simulink model "DualBuckPPS_PI"  (R2024b)
settings: Solver=ode45  StartTime=0.0  StopTime=0.8  RelTol=1e-3
model workspace (MAT data in the model file):
  D = 50
  T = 0.033
  T_pulse = 0.02
undefined symbols (not defined in the file): I_I, I_V, P, P_I, P_V, TP
libraries: spsOnDelayLib x13, spsCurrentMeasurementLib x11, spsSeriesRLCBranchLib x7, dspfdesign x6, spsMosfetLib x4, slpidlib x4, spsVoltageMeasurementLib x4, simulink x3, spsControlledCurrentSourceLib x1, spsDCVoltageSourceLib x1, spspowerguiLib x1
settings Model: SimulationMode=accelerator  Creator=10474  LastModifiedBy=admin
settings SolverCC: AlgebraicLoopSolver=TrustRegion
settings OptimizationCC: ReuseModelBlockBuffer=off
settings DebuggingCC: UnconnectedInputMsg=warning  UnconnectedOutputMsg=warning  UnconnectedLineMsg=warning  ArithmeticOperatorsInVariantConditions=warning
settings ModelReferenceCC: EnableRefExpFcnMdlSchedulingChecks=on
settings SFSimCC: CustomCodeUndefinedFunction=UseInterfaceOnly
settings RTWCC: GPUComputeCapability=3.5
settings CodeAppCC: StateflowObjectComments=on

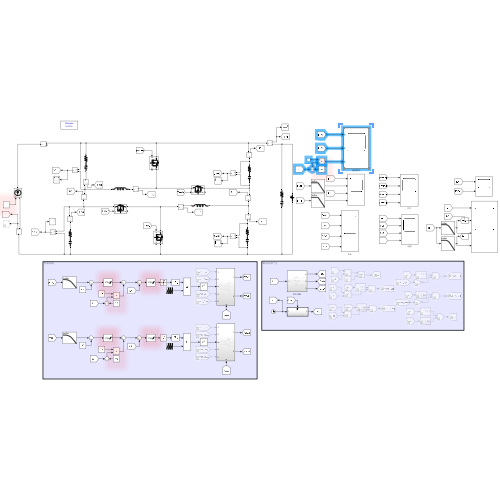
[thumbnail: Simulink's stored preview of the top-level diagram]
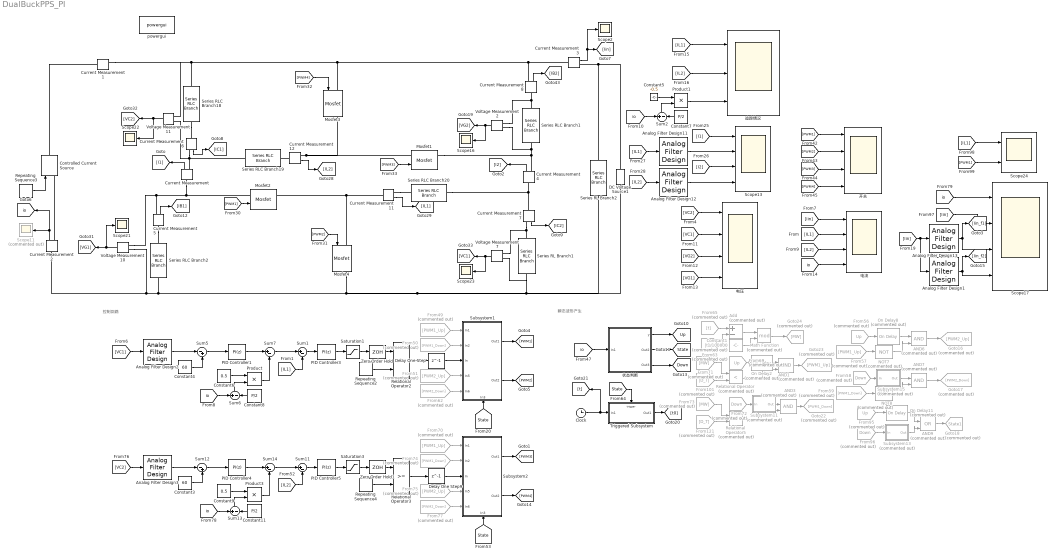
== system DualBuckPPS_PI ==
  note: 控制回路
  note: 瞬态波形产生
  AND{1,3,6..7} (4 alike) : Logic  Commented=on  IconShape=distinctive  AllPortsSameDT=off  OutDataTypeStr=boolean
  AND9 : Logic  Commented=on  Operator=OR  IconShape=distinctive  AllPortsSameDT=off  OutDataTypeStr=boolean
  Add : Sum  Commented=on  Inputs=+-
  Analog Filter Design1 : dspfdesign/Analog Filter Design  method=Butterworth  filttype=Lowpass  N=2  Wlo=2*pi*2500  Whi=80  Rp=2  Rs=40
  Analog Filter Design11 : dspfdesign/Analog Filter Design  method=Butterworth  filttype=Lowpass  N=8  Wlo=2*pi*5000  Whi=80  Rp=2  Rs=40
  Analog Filter Design12 : dspfdesign/Analog Filter Design  method=Butterworth  filttype=Lowpass  N=8  Wlo=2*pi*5000  Whi=80  Rp=2  Rs=40
  Analog Filter Design13 : dspfdesign/Analog Filter Design  method=Butterworth  filttype=Lowpass  N=2  Wlo=2*pi*10000  Whi=80  Rp=2  Rs=40
  Analog Filter Design2 : dspfdesign/Analog Filter Design  method=Butterworth  filttype=Lowpass  N=1  Wlo=10  Whi=80  Rp=2  Rs=40
  Analog Filter Design3 : dspfdesign/Analog Filter Design  method=Butterworth  filttype=Lowpass  N=1  Wlo=10  Whi=80  Rp=2  Rs=40
  Clock : Clock
  Constant1 : Constant  Commented=on  Value=1/100000
  Constant11 : Constant  Value=P/2
  Constant3 : Constant  Value=60
  Constant4 : Constant  Value=60
  Constant5 : Constant  Value=-0.5
  Constant6 : Constant  Value=0.5
  Constant7 : Constant  Value=P/2
  Constant8 : Constant  Value=P/2
  Constant9 : Constant  Value=0.5
  Controlled Current Source : spsControlledCurrentSourceLib/Controlled Current Source  Initialize=on  Source_Type=DC  Amplitude=0  Phase=0  Frequency=0  Measurements=None
  Current Measurement{,1..8,11..12} (11 alike) : spsCurrentMeasurementLib/Current Measurement  PhasorSimulation=off  OutputType=Complex  PSBequivalent=0
  DC Voltage Source1 : spsDCVoltageSourceLib/DC Voltage Source  Amplitude=270  Measurements=None
  Delay One Step : Delay  DelayLength=1
  Delay One Step9 : Delay  DelayLength=1
  From101 : From  Commented=on  GotoTag=D_T
  From121 : From  Commented=on  GotoTag=D_T
  From49 : From  Commented=on  GotoTag=PWM1_Up
  From50 : From  Commented=on  GotoTag=PWM1_Down
  From51 : From  Commented=on  GotoTag=PWM2_Up
  From56 : From  Commented=on  GotoTag=Up  TagVisibility=global
  From57 : From  Commented=on  GotoTag=PWM1_Up
  From58 : From  Commented=on  GotoTag=Down  TagVisibility=global
  From59 : From  Commented=on  GotoTag=PWM1_Down
  From62 : From  Commented=on  GotoTag=PWM2_Down
  From63 : From  Commented=on  GotoTag=t0
  From65 : From  Commented=on  GotoTag=t
  From69 : From  Commented=on  GotoTag=Up  TagVisibility=global
  From70 : From  Commented=on  GotoTag=PWM1_Up
  From71 : From  Commented=on  GotoTag=MW
  From72 : From  Commented=on  GotoTag=Down  TagVisibility=global
  From73 : From  Commented=on  GotoTag=MW
  From74 : From  Commented=on  GotoTag=PWM1_Down
  From75 : From  Commented=on  GotoTag=PWM2_Up
  From77 : From  Commented=on  GotoTag=PWM2_Down
  From95 : From  Commented=on  GotoTag=Up  TagVisibility=global
  From96 : From  Commented=on  GotoTag=Down  TagVisibility=global
  Goto16 : Goto  Commented=on  GotoTag=PWM2_Up
  Goto17 : Goto  Commented=on  GotoTag=PWM2_Down
  Goto18 : Goto  Commented=on  GotoTag=State1  TagVisibility=global
  Goto22 : Goto  Commented=on  GotoTag=PWM1_Down
  Goto23 : Goto  Commented=on  GotoTag=PWM1_Up
  Goto24 : Goto  Commented=on  GotoTag=MW
  Math Function : Math  Commented=on  Operator=mod
  Mosfet{1..4} (4 alike) : spsMosfetLib/Mosfet  Ron=53e-3  Lon=0  Rd=0.001  Vfd=2  IC=0  Rs=1e5  Cs=inf  Measurements=on
  NOT7 : Logic  Commented=on  Operator=NOT  IconShape=distinctive  AllPortsSameDT=off  OutDataTypeStr=boolean
  NOT8 : Logic  Commented=on  Operator=NOT  IconShape=distinctive  AllPortsSameDT=off  OutDataTypeStr=boolean
  On Delay11 : spsOnDelayLib/On Delay  Commented=on  DelayType=Off delay  delay=ceil(TP*1e5)*1e-5-TP  ic=0  Ts=0
  On Delay2 : spsOnDelayLib/On Delay  Commented=on  DelayType=Off delay  delay=ceil(TP*1e5)*1e-5-TP  ic=0  Ts=0
  On Delay8 : spsOnDelayLib/On Delay  Commented=on  DelayType=Off delay  delay=ceil(TP*1e5)*1e-5-TP  ic=0  Ts=0
  PID Controller1 : slpidlib/PID Controller  Controller=PI  Form=Parallel  TimeDomain=Discrete-time  UseExternalTs=off  SampleTime=-1  IntegratorMethod=Forward Euler  FilterMethod=Forward Euler  ControllerParametersSource=internal  P=P_V  I=I_V  UseKiTs=off  D=0  UseExternalDerivativeSource=off  N=100  UseFilter=on  TunerSelectOption=Transfer Function Based (PID Tuner App)  InitialConditionSource=internal  InitialConditionForIntegrator=0  InitialConditionForFilter=0  DifferentiatorICPrevScaledInput=0  ExternalReset=none  TrackingMode=off  Kt=1  LimitOutput=on  SatLimitsSource=internal  UpperSaturationLimit=10  LowerSaturationLimit=-10  LinearizeAsGain=on  AntiWindupMode=none  Kb=1  LimitIntegrator=off  UpperIntegratorSaturationLimit=inf  LowerIntegratorSaturationLimit=-inf  POutMin=[]  POutMax=[]  IOutMin=[]  IOutMax=[]  DOutMin=[]  DOutMax=[]  NOutMin=[]  NOutMax=[]  SumOutMin=[]  SumOutMax=[]  SaturationOutMin=[]  SaturationOutMax=[]  PParamMin=[]  PParamMax=[]  IParamMin=[]  IParamMax=[]  DParamMin=[]  DParamMax=[]  NParamMin=[]  NParamMax=[]  KbParamMin=[]  KbParamMax=[]  KtParamMin=[]  KtParamMax=[]  KbOutMin=[]  KbOutMax=[]  KtOutMin=[]  KtOutMax=[]  IntegratorOutMin=[]  IntegratorOutMax=[]  FilterOutMin=[]  FilterOutMax=[]  SumI1OutMin=[]  SumI1OutMax=[]  SumI2OutMin=[]  SumI2OutMax=[]  SumI3OutMin=[]  SumI3OutMax=[]  SumI4OutMin=[]  SumI4OutMax=[]  SumDOutMin=[]  SumDOutMax=[]  DifferentiatorOutMin=[]  DifferentiatorOutMax=[]  FilterDiffOutCoefMin=[]  FilterDiffOutCoefMax=[]  ReciprocalOutMin=[]  ReciprocalOutMax=[]  SumDenOutMin=[]  SumDenOutMax=[]  SumNumOutMin=[]  SumNumOutMax=[]  DivideOutMin=[]  DivideOutMax=[]  UdiffTsProdOutMin=[]  UdiffTsProdOutMax=[]  NTsProdOutMin=[]  NTsProdOutMax=[]  UintegralTsProdOutMin=[]  UintegralTsProdOutMax=[]  UngainTsProdOutMin=[]  UngainTsProdOutMax=[]  ClampingZeroOutDataTypeStr=Inherit: Inherit via back propagation  ClampingZeroOutMin=[]  ClampingZeroOutMax=[]  FilterDenConstantOutDataTypeStr=Inherit: Inherit via back propagation  FilterDenConstantOutMin=[]  FilterDenConstantOutMax=[]  PCopyOutDataTypeStr=Inherit: Inherit via back propagation  PCopyOutMin=[]  PCopyOutMax=[]  NCopyOutDataTypeStr=Inherit: Inherit via back propagation  NCopyOutMin=[]  NCopyOutMax=[]  IntegratorContinuousStateAttributes=''  IntegratorStateMustResolveToSignalObject=off  IntegratorRTWStateStorageClass=Auto  FilterContinuousStateAttributes=''  FilterStateMustResolveToSignalObject=off  FilterRTWStateStorageClass=Auto  ParallelPVariant=InternalParameters  IdealPVariant=Disabled  IVariant=InternalParameters  DVariant=Disabled  IntegratorVariant=Discrete  SatVariant=Enabled  AWVariant=Passthrough  PCopyVariant=Disabled  TRVariant=Disabled  FdbkBlocksVariant=Forward  IdealPFdbkVariant=Disabled  SatFdbkVariant=Disabled  DerivativeFilterVariant=Disabled  NVariant=Disabled  NCopyVariant=Disabled_SignalSpec  FilterICVariant=Disabled  IntegratorICVariant=InternalICs  ExternalResetVariant=Disabled  TRSumVariant=Passthrough  SumFdbkVariant=Disabled  SumVariant=Sum_PI  TsampFilterVariant=InternalTs  TsampNgainVariant=Passthrough  TsampIntegralVariant=Disabled_SignalSpec  ExternalSaturationOutDataTypeStr=Inherit: Same as second input  DerivativeSourceVariant=Disabled  PreIntVariant=InternalPreInt
  PID Controller3 : slpidlib/PID Controller  Controller=PI  Form=Parallel  TimeDomain=Discrete-time  UseExternalTs=off  SampleTime=-1  IntegratorMethod=Forward Euler  FilterMethod=Forward Euler  ControllerParametersSource=internal  P=P_I  I=I_I  UseKiTs=off  D=0  UseExternalDerivativeSource=off  N=100  UseFilter=on  TunerSelectOption=Transfer Function Based (PID Tuner App)  InitialConditionSource=internal  InitialConditionForIntegrator=0  InitialConditionForFilter=0  DifferentiatorICPrevScaledInput=0  ExternalReset=none  TrackingMode=off  Kt=1  LimitOutput=on  SatLimitsSource=internal  UpperSaturationLimit=0.98  LowerSaturationLimit=0  LinearizeAsGain=on  AntiWindupMode=none  Kb=1  LimitIntegrator=off  UpperIntegratorSaturationLimit=inf  LowerIntegratorSaturationLimit=-inf  POutMin=[]  POutMax=[]  IOutMin=[]  IOutMax=[]  DOutMin=[]  DOutMax=[]  NOutMin=[]  NOutMax=[]  SumOutMin=[]  SumOutMax=[]  SaturationOutMin=[]  SaturationOutMax=[]  PParamMin=[]  PParamMax=[]  IParamMin=[]  IParamMax=[]  DParamMin=[]  DParamMax=[]  NParamMin=[]  NParamMax=[]  KbParamMin=[]  KbParamMax=[]  KtParamMin=[]  KtParamMax=[]  KbOutMin=[]  KbOutMax=[]  KtOutMin=[]  KtOutMax=[]  IntegratorOutMin=[]  IntegratorOutMax=[]  FilterOutMin=[]  FilterOutMax=[]  SumI1OutMin=[]  SumI1OutMax=[]  SumI2OutMin=[]  SumI2OutMax=[]  SumI3OutMin=[]  SumI3OutMax=[]  SumI4OutMin=[]  SumI4OutMax=[]  SumDOutMin=[]  SumDOutMax=[]  DifferentiatorOutMin=[]  DifferentiatorOutMax=[]  FilterDiffOutCoefMin=[]  FilterDiffOutCoefMax=[]  ReciprocalOutMin=[]  ReciprocalOutMax=[]  SumDenOutMin=[]  SumDenOutMax=[]  SumNumOutMin=[]  SumNumOutMax=[]  DivideOutMin=[]  DivideOutMax=[]  UdiffTsProdOutMin=[]  UdiffTsProdOutMax=[]  NTsProdOutMin=[]  NTsProdOutMax=[]  UintegralTsProdOutMin=[]  UintegralTsProdOutMax=[]  UngainTsProdOutMin=[]  UngainTsProdOutMax=[]  ClampingZeroOutDataTypeStr=Inherit: Inherit via back propagation  ClampingZeroOutMin=[]  ClampingZeroOutMax=[]  FilterDenConstantOutDataTypeStr=Inherit: Inherit via back propagation  FilterDenConstantOutMin=[]  FilterDenConstantOutMax=[]  PCopyOutDataTypeStr=Inherit: Inherit via back propagation  PCopyOutMin=[]  PCopyOutMax=[]  NCopyOutDataTypeStr=Inherit: Inherit via back propagation  NCopyOutMin=[]  NCopyOutMax=[]  IntegratorContinuousStateAttributes=''  IntegratorStateMustResolveToSignalObject=off  IntegratorRTWStateStorageClass=Auto  FilterContinuousStateAttributes=''  FilterStateMustResolveToSignalObject=off  FilterRTWStateStorageClass=Auto  ParallelPVariant=InternalParameters  IdealPVariant=Disabled  IVariant=InternalParameters  DVariant=Disabled  IntegratorVariant=Discrete  SatVariant=Enabled  AWVariant=Passthrough  PCopyVariant=Disabled  TRVariant=Disabled  FdbkBlocksVariant=Forward  IdealPFdbkVariant=Disabled  SatFdbkVariant=Disabled  DerivativeFilterVariant=Disabled  NVariant=Disabled  NCopyVariant=Disabled_SignalSpec  FilterICVariant=Disabled  IntegratorICVariant=InternalICs  ExternalResetVariant=Disabled  TRSumVariant=Passthrough  SumFdbkVariant=Disabled  SumVariant=Sum_PI  TsampFilterVariant=InternalTs  TsampNgainVariant=Passthrough  TsampIntegralVariant=Disabled_SignalSpec  ExternalSaturationOutDataTypeStr=Inherit: Same as second input  DerivativeSourceVariant=Disabled  PreIntVariant=InternalPreInt
  PID Controller4 : slpidlib/PID Controller  Controller=PI  Form=Parallel  TimeDomain=Discrete-time  UseExternalTs=off  SampleTime=-1  IntegratorMethod=Forward Euler  FilterMethod=Forward Euler  ControllerParametersSource=internal  P=P_V  I=I_V  UseKiTs=off  D=0  UseExternalDerivativeSource=off  N=100  UseFilter=on  TunerSelectOption=Transfer Function Based (PID Tuner App)  InitialConditionSource=internal  InitialConditionForIntegrator=0  InitialConditionForFilter=0  DifferentiatorICPrevScaledInput=0  ExternalReset=none  TrackingMode=off  Kt=1  LimitOutput=on  SatLimitsSource=internal  UpperSaturationLimit=10  LowerSaturationLimit=-10  LinearizeAsGain=on  AntiWindupMode=none  Kb=1  LimitIntegrator=off  UpperIntegratorSaturationLimit=inf  LowerIntegratorSaturationLimit=-inf  POutMin=[]  POutMax=[]  IOutMin=[]  IOutMax=[]  DOutMin=[]  DOutMax=[]  NOutMin=[]  NOutMax=[]  SumOutMin=[]  SumOutMax=[]  SaturationOutMin=[]  SaturationOutMax=[]  PParamMin=[]  PParamMax=[]  IParamMin=[]  IParamMax=[]  DParamMin=[]  DParamMax=[]  NParamMin=[]  NParamMax=[]  KbParamMin=[]  KbParamMax=[]  KtParamMin=[]  KtParamMax=[]  KbOutMin=[]  KbOutMax=[]  KtOutMin=[]  KtOutMax=[]  IntegratorOutMin=[]  IntegratorOutMax=[]  FilterOutMin=[]  FilterOutMax=[]  SumI1OutMin=[]  SumI1OutMax=[]  SumI2OutMin=[]  SumI2OutMax=[]  SumI3OutMin=[]  SumI3OutMax=[]  SumI4OutMin=[]  SumI4OutMax=[]  SumDOutMin=[]  SumDOutMax=[]  DifferentiatorOutMin=[]  DifferentiatorOutMax=[]  FilterDiffOutCoefMin=[]  FilterDiffOutCoefMax=[]  ReciprocalOutMin=[]  ReciprocalOutMax=[]  SumDenOutMin=[]  SumDenOutMax=[]  SumNumOutMin=[]  SumNumOutMax=[]  DivideOutMin=[]  DivideOutMax=[]  UdiffTsProdOutMin=[]  UdiffTsProdOutMax=[]  NTsProdOutMin=[]  NTsProdOutMax=[]  UintegralTsProdOutMin=[]  UintegralTsProdOutMax=[]  UngainTsProdOutMin=[]  UngainTsProdOutMax=[]  ClampingZeroOutDataTypeStr=Inherit: Inherit via back propagation  ClampingZeroOutMin=[]  ClampingZeroOutMax=[]  FilterDenConstantOutDataTypeStr=Inherit: Inherit via back propagation  FilterDenConstantOutMin=[]  FilterDenConstantOutMax=[]  PCopyOutDataTypeStr=Inherit: Inherit via back propagation  PCopyOutMin=[]  PCopyOutMax=[]  NCopyOutDataTypeStr=Inherit: Inherit via back propagation  NCopyOutMin=[]  NCopyOutMax=[]  IntegratorContinuousStateAttributes=''  IntegratorStateMustResolveToSignalObject=off  IntegratorRTWStateStorageClass=Auto  FilterContinuousStateAttributes=''  FilterStateMustResolveToSignalObject=off  FilterRTWStateStorageClass=Auto  ParallelPVariant=InternalParameters  IdealPVariant=Disabled  IVariant=InternalParameters  DVariant=Disabled  IntegratorVariant=Discrete  SatVariant=Enabled  AWVariant=Passthrough  PCopyVariant=Disabled  TRVariant=Disabled  FdbkBlocksVariant=Forward  IdealPFdbkVariant=Disabled  SatFdbkVariant=Disabled  DerivativeFilterVariant=Disabled  NVariant=Disabled  NCopyVariant=Disabled_SignalSpec  FilterICVariant=Disabled  IntegratorICVariant=InternalICs  ExternalResetVariant=Disabled  TRSumVariant=Passthrough  SumFdbkVariant=Disabled  SumVariant=Sum_PI  TsampFilterVariant=InternalTs  TsampNgainVariant=Passthrough  TsampIntegralVariant=Disabled_SignalSpec  ExternalSaturationOutDataTypeStr=Inherit: Same as second input  DerivativeSourceVariant=Disabled  PreIntVariant=InternalPreInt
  PID Controller5 : slpidlib/PID Controller  Controller=PI  Form=Parallel  TimeDomain=Discrete-time  UseExternalTs=off  SampleTime=-1  IntegratorMethod=Forward Euler  FilterMethod=Forward Euler  ControllerParametersSource=internal  P=P_I  I=I_I  UseKiTs=off  D=0  UseExternalDerivativeSource=off  N=100  UseFilter=on  TunerSelectOption=Transfer Function Based (PID Tuner App)  InitialConditionSource=internal  InitialConditionForIntegrator=0  InitialConditionForFilter=0  DifferentiatorICPrevScaledInput=0  ExternalReset=none  TrackingMode=off  Kt=1  LimitOutput=on  SatLimitsSource=internal  UpperSaturationLimit=0.98  LowerSaturationLimit=0  LinearizeAsGain=on  AntiWindupMode=none  Kb=1  LimitIntegrator=off  UpperIntegratorSaturationLimit=inf  LowerIntegratorSaturationLimit=-inf  POutMin=[]  POutMax=[]  IOutMin=[]  IOutMax=[]  DOutMin=[]  DOutMax=[]  NOutMin=[]  NOutMax=[]  SumOutMin=[]  SumOutMax=[]  SaturationOutMin=[]  SaturationOutMax=[]  PParamMin=[]  PParamMax=[]  IParamMin=[]  IParamMax=[]  DParamMin=[]  DParamMax=[]  NParamMin=[]  NParamMax=[]  KbParamMin=[]  KbParamMax=[]  KtParamMin=[]  KtParamMax=[]  KbOutMin=[]  KbOutMax=[]  KtOutMin=[]  KtOutMax=[]  IntegratorOutMin=[]  IntegratorOutMax=[]  FilterOutMin=[]  FilterOutMax=[]  SumI1OutMin=[]  SumI1OutMax=[]  SumI2OutMin=[]  SumI2OutMax=[]  SumI3OutMin=[]  SumI3OutMax=[]  SumI4OutMin=[]  SumI4OutMax=[]  SumDOutMin=[]  SumDOutMax=[]  DifferentiatorOutMin=[]  DifferentiatorOutMax=[]  FilterDiffOutCoefMin=[]  FilterDiffOutCoefMax=[]  ReciprocalOutMin=[]  ReciprocalOutMax=[]  SumDenOutMin=[]  SumDenOutMax=[]  SumNumOutMin=[]  SumNumOutMax=[]  DivideOutMin=[]  DivideOutMax=[]  UdiffTsProdOutMin=[]  UdiffTsProdOutMax=[]  NTsProdOutMin=[]  NTsProdOutMax=[]  UintegralTsProdOutMin=[]  UintegralTsProdOutMax=[]  UngainTsProdOutMin=[]  UngainTsProdOutMax=[]  ClampingZeroOutDataTypeStr=Inherit: Inherit via back propagation  ClampingZeroOutMin=[]  ClampingZeroOutMax=[]  FilterDenConstantOutDataTypeStr=Inherit: Inherit via back propagation  FilterDenConstantOutMin=[]  FilterDenConstantOutMax=[]  PCopyOutDataTypeStr=Inherit: Inherit via back propagation  PCopyOutMin=[]  PCopyOutMax=[]  NCopyOutDataTypeStr=Inherit: Inherit via back propagation  NCopyOutMin=[]  NCopyOutMax=[]  IntegratorContinuousStateAttributes=''  IntegratorStateMustResolveToSignalObject=off  IntegratorRTWStateStorageClass=Auto  FilterContinuousStateAttributes=''  FilterStateMustResolveToSignalObject=off  FilterRTWStateStorageClass=Auto  ParallelPVariant=InternalParameters  IdealPVariant=Disabled  IVariant=InternalParameters  DVariant=Disabled  IntegratorVariant=Discrete  SatVariant=Enabled  AWVariant=Passthrough  PCopyVariant=Disabled  TRVariant=Disabled  FdbkBlocksVariant=Forward  IdealPFdbkVariant=Disabled  SatFdbkVariant=Disabled  DerivativeFilterVariant=Disabled  NVariant=Disabled  NCopyVariant=Disabled_SignalSpec  FilterICVariant=Disabled  IntegratorICVariant=InternalICs  ExternalResetVariant=Disabled  TRSumVariant=Passthrough  SumFdbkVariant=Disabled  SumVariant=Sum_PI  TsampFilterVariant=InternalTs  TsampNgainVariant=Passthrough  TsampIntegralVariant=Disabled_SignalSpec  ExternalSaturationOutDataTypeStr=Inherit: Same as second input  DerivativeSourceVariant=Disabled  PreIntVariant=InternalPreInt
  Product : Product
  Product1 : Product
  Product3 : Product
  Relational Operator : RelationalOperator  Commented=on  Operator=<  OutDataTypeStr=boolean  RndMeth=Simplest  InputSameDT=off
  Relational Operator2 : RelationalOperator  OutDataTypeStr=boolean  RndMeth=Simplest  InputSameDT=off
  Relational Operator3 : RelationalOperator  OutDataTypeStr=boolean  RndMeth=Simplest  InputSameDT=off
  Relational Operator5 : RelationalOperator  Commented=on  Operator=<  OutDataTypeStr=boolean  RndMeth=Simplest  InputSameDT=off
  Repeating Sequence2 : simulink/Sources/Repeating Sequence  rep_seq_t=[0 1/100000]  rep_seq_y=[0 1]
  Repeating Sequence3 : simulink/Sources/Repeating Sequence  rep_seq_t=[0 TP T_pulse/2+TP T_pulse/2+2*TP T_pulse]  rep_seq_y=[0 P P 0 0]
  Repeating Sequence4 : simulink/Sources/Repeating Sequence  rep_seq_t=[0 1/100000]  rep_seq_y=[0 1]
  Saturation1 : Saturate  UpperLimit=0.98  LowerLimit=0
  Saturation3 : Saturate  UpperLimit=0.98  LowerLimit=0
  Scope11 : Scope  Commented=on
  Scope13 : Scope  NumInputPorts=4
  Scope{2,16,21..23} (5 alike) : Scope
  Scope17 : Scope  NumInputPorts=4
  Scope24 : Scope  NumInputPorts=2
  Series RL Branch1 : spsSeriesRLCBranchLib/Series RLC Branch  LConnTagsString=__new0  RConnTagsString=__new0  BranchType=RC  Resistance=0.001  Inductance=1e-3  SetiL0=off  InitialCurrent=0  Capacitance=1e-6  Setx0=on  InitialVoltage=12  Measurements=None
  Series RL Branch2 : spsSeriesRLCBranchLib/Series RLC Branch  LConnTagsString=__new0  RConnTagsString=__new0  BranchType=RC  Resistance=0.001  Inductance=1e-3  SetiL0=off  InitialCurrent=0  Capacitance=100e-6  Setx0=on  InitialVoltage=270  Measurements=None
  Series RLC Branch1 : spsSeriesRLCBranchLib/Series RLC Branch  LConnTagsString=__new0  RConnTagsString=__new0  BranchType=RC  Resistance=0.001  Inductance=1e-3  SetiL0=off  InitialCurrent=0  Capacitance=2.48e-3  Setx0=on  InitialVoltage=12  Measurements=None
  Series RLC Branch18 : spsSeriesRLCBranchLib/Series RLC Branch  LConnTagsString=__new0  RConnTagsString=__new0  BranchType=RC  Resistance=0.001  Inductance=1e-3  SetiL0=off  InitialCurrent=0  Capacitance=1e-6  Setx0=on  InitialVoltage=12  Measurements=None
  Series RLC Branch19 : spsSeriesRLCBranchLib/Series RLC Branch  LConnTagsString=__new0  RConnTagsString=__new0  BranchType=L  Resistance=0.01  Inductance=260e-6  SetiL0=off  InitialCurrent=15  Capacitance=1e-3  Setx0=off  InitialVoltage=0  Measurements=None
  Series RLC Branch2 : spsSeriesRLCBranchLib/Series RLC Branch  LConnTagsString=__new0  RConnTagsString=__new0  BranchType=RC  Resistance=0.2  Inductance=1e-3  SetiL0=off  InitialCurrent=0  Capacitance=2.48e-3  Setx0=on  InitialVoltage=12  Measurements=None
  Series RLC Branch20 : spsSeriesRLCBranchLib/Series RLC Branch  LConnTagsString=__new0  RConnTagsString=__new0  BranchType=L  Resistance=0.01  Inductance=260e-6  SetiL0=off  InitialCurrent=5  Capacitance=1e-3  Setx0=off  InitialVoltage=0  Measurements=None
  Subsystem1 : Subsystem
      settings: PortSchema="{\"entries\":[{\"content\":{\"sides\":[{\"content\":{\"connectorIds\":[\"In1\",\"In2\",\"In3\",\"In4\",\"In5\"]},\"type\":\"ConnectorPlacement.EquallySpacedRectSide\",\"uuid\":\"12f56cea-dd87-479d-8ac5-f677a0a856ab\"},{\"content\":{\"connectorIds\":[\"Out1\",\"Out2\"],\"side\":\"RIGHT\"},\"type\":\"ConnectorPlacement.EquallySpacedRectSide\",\"uuid\":\"93daadb0-c8ef-4d9e-87ae-a550f970c223\"},{\"content\":{\"side\":\"TOP\"},\"type\":\"ConnectorPlacement.EquallySpacedRectSide\",\"uuid\":\"18f26d28-3d48-45f0-84e1-51e7663a8b99\"},{\"content\":{\"connectorIds\":[\"In6\"],\"side\":\"BOTTOM\"},\"type\":\"ConnectorPlacement.EquallySpacedRectSide\",\"uuid\":\"53ae5f66-9a34-49e2-9ad8-502cdcf805c1\"}]},\"type\":\"ConnectorPlacement.EquallySpacedConnector\",\"uuid\":\"751889f7-46a5-4d64-ba57-d2d7ffe777e8\"}],\"packageUris\":[\"http://schema.mathworks.com/mf0/Connector/R2020b\"],\"version\":\"1.0\"}"
  Subsystem11 : Subsystem  Commented=on
  Subsystem13 : Subsystem  Commented=on
  Subsystem15 : Subsystem  Commented=on
  Subsystem2 : Subsystem
      settings: PortSchema="{\"entries\":[{\"content\":{\"sides\":[{\"content\":{\"connectorIds\":[\"In1\",\"In2\",\"In3\",\"In4\",\"In5\"]},\"type\":\"ConnectorPlacement.EquallySpacedRectSide\",\"uuid\":\"12f56cea-dd87-479d-8ac5-f677a0a856ab\"},{\"content\":{\"connectorIds\":[\"Out1\",\"Out2\"],\"side\":\"RIGHT\"},\"type\":\"ConnectorPlacement.EquallySpacedRectSide\",\"uuid\":\"93daadb0-c8ef-4d9e-87ae-a550f970c223\"},{\"content\":{\"side\":\"TOP\"},\"type\":\"ConnectorPlacement.EquallySpacedRectSide\",\"uuid\":\"18f26d28-3d48-45f0-84e1-51e7663a8b99\"},{\"content\":{\"connectorIds\":[\"In6\"],\"side\":\"BOTTOM\"},\"type\":\"ConnectorPlacement.EquallySpacedRectSide\",\"uuid\":\"53ae5f66-9a34-49e2-9ad8-502cdcf805c1\"}]},\"type\":\"ConnectorPlacement.EquallySpacedConnector\",\"uuid\":\"751889f7-46a5-4d64-ba57-d2d7ffe777e8\"}],\"packageUris\":[\"http://schema.mathworks.com/mf0/Connector/R2020b\"],\"version\":\"1.0\"}"
  Sum{1,7,11,14} (4 alike) : Sum  Inputs=|+-
  Sum12 : Sum  Inputs=|-+
  Sum13 : Sum  Inputs=+-
  Sum2 : Sum  Inputs=+-
  Sum5 : Sum  Inputs=|-+
  Sum6 : Sum  Inputs=+-
  Triggered Subsystem : Subsystem  TreatAsAtomicUnit=on
  Voltage Measurement{2,7,10..11} (4 alike) : spsVoltageMeasurementLib/Voltage Measurement  PhasorSimulation=off  OutputType=Complex  PSBequivalent=0
  Zero-Order Hold : ZeroOrderHold  SampleTime=1e-5
  Zero-Order Hold1 : ZeroOrderHold  SampleTime=1e-5
  powergui : spspowerguiLib/powergui  Priority=1  SimulationMode=Discrete  SampleTime=1e-7  frequency=60  Iterations=50  frequencyindice=0  Pbase=100e6  ErrMax=1e-4  UnitsV=kV  UnitsW=MW  buscounter=0  FunctionMessages=off  echomessages=off  EnableUseOfTLC=off  CurrentSourceSwitches=off  DisableSnubberDevices=off  DisableRonSwitches=off  DisableVfSwitches=off  DisplayEquations=off  AutomaticDiscreteSolvers=off  SolverType=Tustin/Backward Euler (TBE)  Interpol=off  ExternalGateDelay=off  methode=off  Ts=100  x0status=blocks  SPID=on  SwTol=0  HookPort=off  NonlinearTolerance=1e-4  nMaxIteration=100  ContinueOnMaxIteration=off  RestoreLinks=warning  ResistiveCurrentMeasurement=off  Frange=[0:2:500]  Ylog=off  Xlog=on  ShowGrid=off  save=off  variable=ZData  structure=0  ZoomFFT=off  StartTime=0.0  cycles=1  DisplayStyle=1  fundamental=60  FreqAxis=off  MaxFrequency=1000  frequencyindicesteady=1  RmsSteady=1  display=off
  开关 : Scope  NumInputPorts=4
  状态判断 : Subsystem
  电压 : Scope  NumInputPorts=4
  电流 : Scope  NumInputPorts=4
  追踪情况 : Scope  NumInputPorts=3
  tag scope: Down=global, State=global, Up=global, io=global
  wires:
  [PWM2] -> Mosfet4/1
  Current Measurement12/1 -> [IL2]
  [PWM4] -> Mosfet3/1
  Current Measurement11/1 -> [IL1]
  Voltage Measurement10/1 -> Scope21/1, [VG1]
  [PWM1] -> Mosfet2/1
  Voltage Measurement11/1 -> Scope22/1, [VC2]
  Current Measurement8/1 -> [IB2]
  Current Measurement2/1 -> Scope11/1, [io]
  [VC1] -> Analog Filter Design2/1
  Analog Filter Design2/1 -> Sum5/1
  Sum5/1 -> PID Controller1/1
  Repeating Sequence2/1 -> Relational Operator2/2
  Constant4/1 -> Sum5/2
  [PWM3] -> Mosfet1/1
  Current Measurement3/1 -> Scope2/1, [Iin]
  PID Controller3/1 -> Saturation1/1
  Sum1/1 -> PID Controller3/1
  [io] -> Sum6/1
  Sum6/1 -> Product/2
  Product/1 -> Sum7/2
  Constant6/1 -> Product/1
  [IL1] -> Sum1/2
  Constant8/1 -> Sum6/2
  Current Measurement/1 -> [I1]
  Current Measurement4/1 -> [I2]
  Current Measurement6/1 -> [IC1]
  Current Measurement7/1 -> [IC2]
  [I1] -> Scope13/1
  [I2] -> Scope13/3
  Analog Filter Design11/1 -> Scope13/2
  Analog Filter Design12/1 -> Scope13/4
  Repeating Sequence3/1 -> Controlled Current Source/1
  From57/1 -> NOT7/1
  NOT7/1 -> AND6/2
  AND7/1 -> Goto17/1
  NOT8/1 -> AND7/2
  From59/1 -> NOT8/1
  AND6/1 -> Goto16/1
  [io] -> 状态判断/1(In1)
  状态判断/2(Out2) -> [State]
  状态判断/3(Out3) -> [Down]
  Current Measurement5/1 -> [IB1]
  [IL2] -> Analog Filter Design12/1
  [IL1] -> Analog Filter Design11/1
  [Iin] -> 电流/1
  [IL1] -> 电流/2
  [IL2] -> 电流/3
  [io] -> 电流/4
  Voltage Measurement7/1 -> Scope23/1, [VC1]
  Voltage Measurement2/1 -> [VG2], Scope16/1
  Subsystem1/2(Out2) -> [PWM2]
  From62/1 -> Subsystem1/5(In6)
  From51/1 -> Subsystem1/4(In5)
  [State] -> Subsystem1/6(In3)
  From50/1 -> Subsystem1/2(In2)
  From49/1 -> Subsystem1/1(In1)
  Subsystem1/1(Out1) -> [PWM1]
  [State] -> Triggered Subsystem/Trigger
  Triggered Subsystem/1(Out1) -> [t0]
  From63/1 -> Add/2
  From65/1 -> Add/1
  Add/1 -> Math Function/1
  Constant1/1 -> Math Function/2
  AND1/1 -> Goto23/1
  Math Function/1 -> Goto24/1
  From71/1 -> Relational Operator/1
  From73/1 -> Relational Operator5/1
  Relational Operator5/1 -> AND3/2
  Saturation3/1 -> Zero-Order Hold1/1
  Subsystem2/1(Out1) -> [PWM3]
  From70/1 -> Subsystem2/1(In1)
  From74/1 -> Subsystem2/2(In2)
  [State] -> Subsystem2/6(In3)
  From75/1 -> Subsystem2/4(In5)
  From77/1 -> Subsystem2/5(In6)
  Subsystem2/2(Out2) -> [PWM4]
  Constant11/1 -> Sum13/2
  [IL2] -> Sum11/2
  Constant9/1 -> Product3/1
  Product3/1 -> Sum14/2
  Sum13/1 -> Product3/2
  Sum14/1 -> Sum11/1
  [io] -> Sum13/1
  PID Controller4/1 -> Sum14/1
  Sum11/1 -> PID Controller5/1
  PID Controller5/1 -> Saturation3/1
  Constant3/1 -> Sum12/2
  Repeating Sequence4/1 -> Relational Operator3/2
  Sum12/1 -> PID Controller4/1
  Analog Filter Design3/1 -> Sum12/1
  [VC2] -> Analog Filter Design3/1
  Analog Filter Design13/1 -> Scope17/3, [Iin_f1]
  [Iin] -> Analog Filter Design1/1, Analog Filter Design13/1
  Saturation1/1 -> Zero-Order Hold/1
  Zero-Order Hold/1 -> Relational Operator2/1
  Zero-Order Hold1/1 -> Relational Operator3/1
  状态判断/1(y) -> [Up]
  [io] -> Scope17/1
  Analog Filter Design1/1 -> Scope17/4, [Iin_f2]
  From95/1 -> On Delay11/1
  On Delay11/1 -> AND9/1
  AND9/1 -> Goto18/1
  Relational Operator/1 -> AND1/2
  From56/1 -> On Delay8/1
  On Delay8/1 -> AND6/1
  Relational Operator2/1 -> Delay One Step/1
  Delay One Step/1 -> Subsystem1/3(In)
  Relational Operator3/1 -> Delay One Step9/1
  Delay One Step9/1 -> Subsystem2/3(In)
  AND3/1 -> Goto22/1
  Subsystem15/1(Out) -> AND7/1
  From58/1 -> Subsystem15/1(In)
  From96/1 -> Subsystem13/1(In)
  Subsystem13/1(Out) -> AND9/2
  [Iin] -> Scope17/2
  From101/1 -> Relational Operator/2
  From121/1 -> Relational Operator5/2
  [IL1] -> Scope24/1
  [PWM1] -> Scope24/2
  From69/1 -> On Delay2/1
  On Delay2/1 -> AND1/1
  From72/1 -> Subsystem11/1(In)
  Subsystem11/1(Out) -> AND3/1
  [VC2] -> 电压/1
  [VC1] -> 电压/2
  [VG2] -> 电压/3
  [VG1] -> 电压/4
  [PWM1] -> 开关/1
  [PWM2] -> 开关/2
  [PWM3] -> 开关/3
  [PWM4] -> 开关/4
  PID Controller1/1 -> Sum7/1
  Sum7/1 -> Sum1/1
  Clock/1 -> [t], Triggered Subsystem/1(In1)
  Constant7/1 -> Sum2/2
  Sum2/1 -> Product1/2
  [io] -> Sum2/1
  Product1/1 -> 追踪情况/3
  Constant5/1 -> Product1/1
  [IL2] -> 追踪情况/2
  [IL1] -> 追踪情况/1
  connections:
  Voltage Measurement10/LConn2 -- Series RL Branch1/RConn1 -- Voltage Measurement7/LConn2 -- DC Voltage Source1/LConn1 -- Series RL Branch2/RConn1 -- Mosfet4/RConn1 -- Series RLC Branch2/RConn1 -- Current Measurement2/LConn1
  Current Measurement3/LConn1 -- Current Measurement1/RConn1 -- Voltage Measurement11/LConn1 -- Series RLC Branch18/LConn1 -- Mosfet3/LConn1 -- Current Measurement8/RConn1
  Current Measurement12/RConn1 -- Mosfet1/LConn1 -- Mosfet3/RConn1
  Current Measurement11/RConn1 -- Series RLC Branch20/LConn1
  Series RLC Branch20/RConn1 -- Current Measurement7/LConn1 -- Current Measurement4/LConn1
  Current Measurement12/LConn1 -- Series RLC Branch19/RConn1
  Series RLC Branch19/LConn1 -- Voltage Measurement11/LConn2 -- Current Measurement/RConn1 -- Current Measurement6/RConn1
  Series RLC Branch1/LConn1 -- Current Measurement8/LConn1 -- Voltage Measurement2/LConn1
  Current Measurement2/RConn1 -- Controlled Current Source/LConn1
  Current Measurement1/LConn1 -- Controlled Current Source/RConn1
  Series RL Branch2/LConn1 -- Current Measurement3/RConn1 -- DC Voltage Source1/RConn1
  Current Measurement5/LConn1 -- Series RLC Branch2/LConn1
  Current Measurement4/RConn1 -- Mosfet1/RConn1 -- Voltage Measurement2/LConn2 -- Series RLC Branch1/RConn1
  Current Measurement7/RConn1 -- Series RL Branch1/LConn1 -- Voltage Measurement7/LConn1
  Series RLC Branch18/RConn1 -- Current Measurement6/LConn1
  Mosfet4/LConn1 -- Current Measurement11/LConn1 -- Mosfet2/RConn1
  Current Measurement/LConn1 -- Voltage Measurement10/LConn1 -- Current Measurement5/RConn1 -- Mosfet2/LConn1

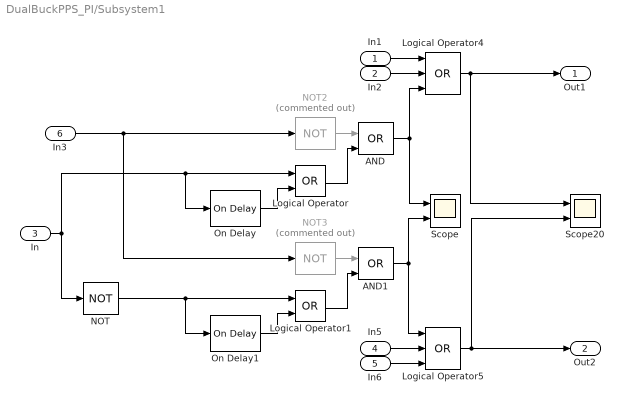
== system DualBuckPPS_PI/Subsystem1 ==
  In1 : Inport
  In2 : Inport  Port=2
  In : Inport  Port=3
  In5 : Inport  Port=4
  In6 : Inport  Port=5
  In3 : Inport  Port=6
  AND : Logic  Operator=OR  IconShape=distinctive  AllPortsSameDT=off  OutDataTypeStr=boolean
  AND1 : Logic  Operator=OR  IconShape=distinctive  AllPortsSameDT=off  OutDataTypeStr=boolean
  Logical Operator : Logic  Operator=OR  AllPortsSameDT=off  OutDataTypeStr=boolean
  Logical Operator1 : Logic  Operator=OR  AllPortsSameDT=off  OutDataTypeStr=boolean
  Logical Operator4 : Logic  Operator=OR  Inputs=3  AllPortsSameDT=off  OutDataTypeStr=boolean
  Logical Operator5 : Logic  Operator=OR  Inputs=3  AllPortsSameDT=off  OutDataTypeStr=boolean
  NOT : Logic  Operator=NOT  IconShape=distinctive  AllPortsSameDT=off  OutDataTypeStr=boolean
  NOT2 : Logic  Commented=on  Operator=NOT  IconShape=distinctive  AllPortsSameDT=off  OutDataTypeStr=boolean
  NOT3 : Logic  Commented=on  Operator=NOT  IconShape=distinctive  AllPortsSameDT=off  OutDataTypeStr=boolean
  On Delay : spsOnDelayLib/On Delay  DelayType=On delay  delay=100e-9  ic=0  Ts=0
  On Delay1 : spsOnDelayLib/On Delay  DelayType=On delay  delay=100e-9  ic=0  Ts=0
  Scope : Scope  NumInputPorts=2
  Scope20 : Scope  NumInputPorts=2
  Out1 : Outport
  Out2 : Outport  Port=2
  wires:
  In5/1 -> Logical Operator5/2
  In6/1 -> Logical Operator5/3
  In3/1 -> NOT3/1, NOT2/1
  In/1 -> Logical Operator/1, On Delay/1, NOT/1
  NOT2/1 -> AND/1
  NOT3/1 -> AND1/1
  Logical Operator1/1 -> AND1/2
  NOT/1 -> Logical Operator1/1, On Delay1/1
  Logical Operator5/1 -> Scope20/2, Out2/1
  Logical Operator4/1 -> Scope20/1, Out1/1
  In2/1 -> Logical Operator4/2
  On Delay/1 -> Logical Operator/2
  On Delay1/1 -> Logical Operator1/2
  AND1/1 -> Scope/2, Logical Operator5/1
  AND/1 -> Logical Operator4/3, Scope/1
  Logical Operator/1 -> AND/2
  In1/1 -> Logical Operator4/1

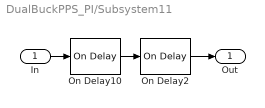
== system DualBuckPPS_PI/Subsystem11 ==
  In : Inport
  On Delay10 : spsOnDelayLib/On Delay  DelayType=On delay  delay=ceil(TP*1e5)*1e-5-TP  ic=0  Ts=0
  On Delay2 : spsOnDelayLib/On Delay  DelayType=Off delay  delay=ceil((TP-(ceil(TP*1e5)*1e-5-TP))*1e5)*1e-5-(TP-(ceil(TP*1e5)*1e-5-TP))  ic=0  Ts=0
  Out : Outport
  wires:
  On Delay2/1 -> Out/1
  In/1 -> On Delay10/1
  On Delay10/1 -> On Delay2/1

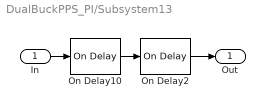
== system DualBuckPPS_PI/Subsystem13 ==
  In : Inport
  On Delay10 : spsOnDelayLib/On Delay  DelayType=On delay  delay=ceil(TP*1e5)*1e-5-TP  ic=0  Ts=0
  On Delay2 : spsOnDelayLib/On Delay  DelayType=Off delay  delay=ceil((TP-(ceil(TP*1e5)*1e-5-TP))*1e5)*1e-5-(TP-(ceil(TP*1e5)*1e-5-TP))  ic=0  Ts=0
  Out : Outport
  wires:
  On Delay10/1 -> On Delay2/1
  In/1 -> On Delay10/1
  On Delay2/1 -> Out/1

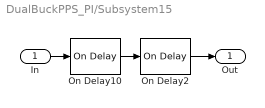
== system DualBuckPPS_PI/Subsystem15 ==
  In : Inport
  On Delay10 : spsOnDelayLib/On Delay  DelayType=On delay  delay=ceil(TP*1e5)*1e-5-TP  ic=0  Ts=0
  On Delay2 : spsOnDelayLib/On Delay  DelayType=Off delay  delay=ceil((TP-(ceil(TP*1e5)*1e-5-TP))*1e5)*1e-5-(TP-(ceil(TP*1e5)*1e-5-TP))  ic=0  Ts=0
  Out : Outport
  wires:
  On Delay10/1 -> On Delay2/1
  In/1 -> On Delay10/1
  On Delay2/1 -> Out/1

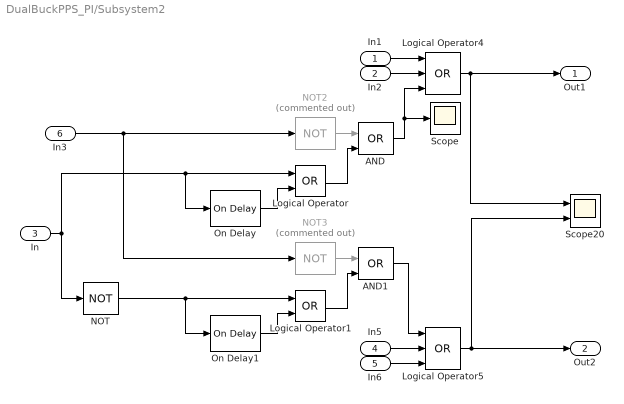
== system DualBuckPPS_PI/Subsystem2 ==
  In1 : Inport
  In2 : Inport  Port=2
  In : Inport  Port=3
  In5 : Inport  Port=4
  In6 : Inport  Port=5
  In3 : Inport  Port=6
  AND : Logic  Operator=OR  IconShape=distinctive  AllPortsSameDT=off  OutDataTypeStr=boolean
  AND1 : Logic  Operator=OR  IconShape=distinctive  AllPortsSameDT=off  OutDataTypeStr=boolean
  Logical Operator : Logic  Operator=OR  AllPortsSameDT=off  OutDataTypeStr=boolean
  Logical Operator1 : Logic  Operator=OR  AllPortsSameDT=off  OutDataTypeStr=boolean
  Logical Operator4 : Logic  Operator=OR  Inputs=3  AllPortsSameDT=off  OutDataTypeStr=boolean
  Logical Operator5 : Logic  Operator=OR  Inputs=3  AllPortsSameDT=off  OutDataTypeStr=boolean
  NOT : Logic  Operator=NOT  IconShape=distinctive  AllPortsSameDT=off  OutDataTypeStr=boolean
  NOT2 : Logic  Commented=on  Operator=NOT  IconShape=distinctive  AllPortsSameDT=off  OutDataTypeStr=boolean
  NOT3 : Logic  Commented=on  Operator=NOT  IconShape=distinctive  AllPortsSameDT=off  OutDataTypeStr=boolean
  On Delay : spsOnDelayLib/On Delay  DelayType=On delay  delay=100e-9  ic=0  Ts=0
  On Delay1 : spsOnDelayLib/On Delay  DelayType=On delay  delay=100e-9  ic=0  Ts=0
  Scope : Scope
  Scope20 : Scope  NumInputPorts=2
  Out1 : Outport
  Out2 : Outport  Port=2
  wires:
  In1/1 -> Logical Operator4/1
  Logical Operator/1 -> AND/2
  AND/1 -> Scope/1, Logical Operator4/3
  AND1/1 -> Logical Operator5/1
  On Delay1/1 -> Logical Operator1/2
  On Delay/1 -> Logical Operator/2
  In2/1 -> Logical Operator4/2
  Logical Operator4/1 -> Out1/1, Scope20/1
  Logical Operator5/1 -> Out2/1, Scope20/2
  NOT/1 -> On Delay1/1, Logical Operator1/1
  Logical Operator1/1 -> AND1/2
  NOT3/1 -> AND1/1
  NOT2/1 -> AND/1
  In/1 -> NOT/1, On Delay/1, Logical Operator/1
  In3/1 -> NOT2/1, NOT3/1
  In6/1 -> Logical Operator5/3
  In5/1 -> Logical Operator5/2

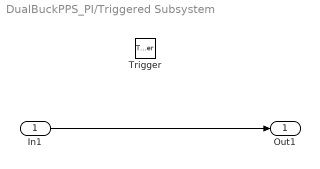
== system DualBuckPPS_PI/Triggered Subsystem ==
  In1 : Inport
  Trigger : TriggerPort  VariantControl=(inherit)
  Out1 : Outport
  wires:
  In1/1 -> Out1/1

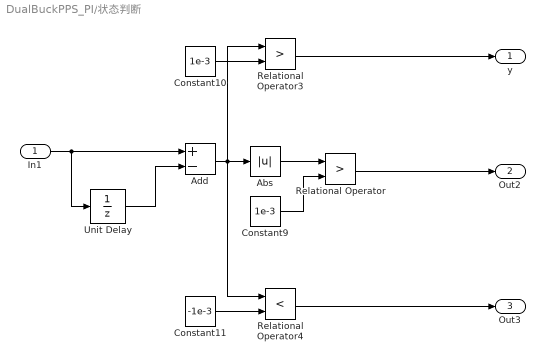
== system DualBuckPPS_PI/状态判断 ==
  In1 : Inport
  Abs : Abs  SaturateOnIntegerOverflow=off
  Add : Sum  Inputs=+-
  Constant10 : Constant  Value=1e-3
  Constant11 : Constant  Value=-1e-3
  Constant9 : Constant  Value=1e-3
  Relational Operator : RelationalOperator  Operator=>  OutDataTypeStr=boolean  RndMeth=Simplest  InputSameDT=off
  Relational Operator3 : RelationalOperator  Operator=>  OutDataTypeStr=boolean  RndMeth=Simplest  InputSameDT=off
  Relational Operator4 : RelationalOperator  Operator=<  OutDataTypeStr=boolean  RndMeth=Simplest  InputSameDT=off
  Unit Delay : UnitDelay  SampleTime=-1  HasFrameUpgradeWarning=on
  y : Outport
  Out2 : Outport  Port=2
  Out3 : Outport  Port=3
  wires:
  In1/1 -> Unit Delay/1, Add/1
  Constant10/1 -> Relational Operator3/2
  Unit Delay/1 -> Add/2
  Constant9/1 -> Relational Operator/2
  Constant11/1 -> Relational Operator4/2
  Add/1 -> Relational Operator4/1, Relational Operator3/1, Abs/1
  Abs/1 -> Relational Operator/1
  Relational Operator3/1 -> y/1
  Relational Operator/1 -> Out2/1
  Relational Operator4/1 -> Out3/1
